simulink library "lib_vehicle_dyn"  (R2024b)
settings: Solver=VariableStepAuto  StartTime=0.0  StopTime=10.0  RelTol=1e-3
undefined symbols (not defined in the file): D
libraries: cstextras x3, simulink x1
settings Model: Creator=simon  LastModifiedBy=simon
settings RTWCC: GPUComputeCapability=3.5

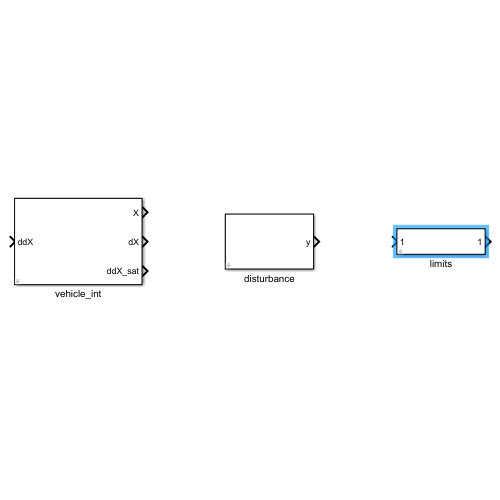
[thumbnail: Simulink's stored preview of the top-level diagram]
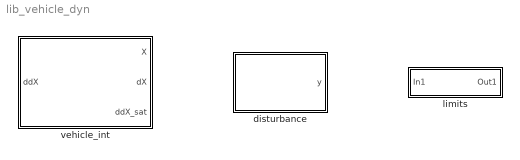
== system lib_vehicle_dyn ==
  disturbance : Subsystem  mask{wn_amp=0, wn_smpl_time=0, wn_gain=0, pg_amp=0, pg_period=0, pg_pw=0, pg_gain=0}
      mask prompts: wn_amp "White noise amplitude"; wn_smpl_time "White noise sampling time"; wn_gain "White noise gain"; pg_amp "Pulse generator amplitude"; pg_period "Pulse generator period"; pg_pw "Pulse generator pulse width [%]"; pg_gain "Pulse generator gain"
      mask DialogControl Control2 Prompt: Disturbance
  limits : Subsystem  mask{satur=0, slew_rate=0, omega=0}
      mask prompts: satur "saturation"
      mask DialogControl Control2 Prompt: Limits
  vehicle_int : Subsystem  mask{x0=0, y0=0, dx0=0, dy0=0, u_sat=0}
      mask DialogControl Control2 Prompt: Vehicle dynamics 2D model

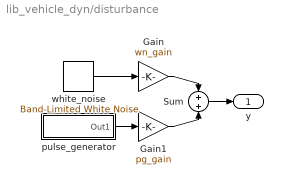
== system lib_vehicle_dyn/disturbance ==
  Gain : Gain  Gain=wn_gain
  Gain1 : Gain  Gain=pg_gain
  Sum : Sum
  pulse_generator : Subsystem
  white_noise : simulink/Sources/Band-Limited White Noise  Cov=wn_amp  Ts=wn_smpl_time  seed=[23341]
  y : Outport
  wires:
  pulse_generator/1(Out1) -> Gain1/1
  white_noise/1 -> Gain/1
  Sum/1 -> y/1
  Gain1/1 -> Sum/2
  Gain/1 -> Sum/1

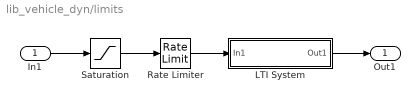
== system lib_vehicle_dyn/limits ==
  In1 : Inport
  LTI System : Subsystem  AncestorBlock=cstblocks/LTI System  BlockChoice=CSS  mask(LTI Block){sys=tf(omega,[1 omega]), IC=[], PadeOrder=0}
      mask prompts: sys "Control:simulink:LTIMaskLabel1"; IC "Control:simulink:LTIMaskLabel2"; PadeOrder "Simulink:blkprm_prompts:TransDelayPadeOrder"
      mask help: Control:simulink:LTIMaskDescription
      mask init:
      | try
      |    % read data to initialize mask variables
      |    [D,Ts,Tdi,Tdo,Tdio,x0,sysname]=...
      |       ltimask('Initialize',gcb,sys,IC);
      |    % update contents
      |    model = bdroot;
      |    df = get_param(model,'dirty');
      |    ltimask('UpdateDiagram',gcb,D,Ts,Tdio,PadeOrder);
      |    try      
      |       % Attempt to modify locked library -> error
      |       % Makes block show ??? when loading CSTBLOCKS
      |       % for the first time
      |       set_param(model,'dirty',df)
      |    end
      | catch ME
      |    sys = [];  IC = [];   sysname = '???';
      |    throw(ME)
      | end
      mask Help: eval('helpview(''control'',''ltisystemblock'');')
      mask Callback sys: ltimask('MaskLTICallback',gcb);
      mask DialogControl sys Prompt: LTI system variable
      mask DialogControl IC Prompt: Initial states (state-space only)
      mask DialogControl PadeOrder Prompt: Pade order (for linearization):
      mask Display: disp(sysname)
  Rate Limiter : RateLimiter  RisingSlewLimit=slew_rate  FallingSlewLimit=-slew_rate  SampleTimeMode=inherited
  Saturation : Saturate  UpperLimit=satur  LowerLimit=-satur
  Out1 : Outport
  wires:
  In1/1 -> Saturation/1
  Saturation/1 -> Rate Limiter/1
  LTI System/1(Out1) -> Out1/1
  Rate Limiter/1 -> LTI System/1(In1)

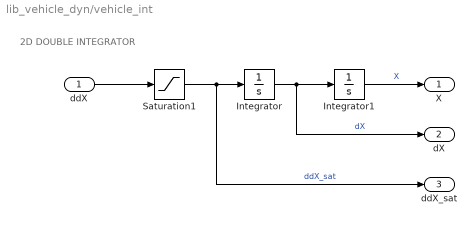
== system lib_vehicle_dyn/vehicle_int ==
  note: 2D DOUBLE INTEGRATOR
  ddX : Inport
  Integrator : Integrator  InitialCondition=[dx0 dy0]
  Integrator1 : Integrator  InitialCondition=[x0 y0]
  Saturation1 : Saturate  UpperLimit=u_sat  LowerLimit=-u_sat
  X : Outport
  dX : Outport  Port=2
  ddX_sat : Outport  Port=3
  wires:
  Saturation1/1 -> ddX_sat/1, Integrator/1  "ddX_sat"
  Integrator/1 -> dX/1, Integrator1/1  "dX"
  ddX/1 -> Saturation1/1
  Integrator1/1 -> X/1  "X"

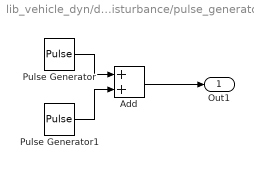
== system lib_vehicle_dyn/disturbance/pulse_generator ==
  Add : Sum
  Pulse Generator : DiscretePulseGenerator  PulseType=Time based  Amplitude=pg_amp  Period=pg_period  PulseWidth=pg_pw
  Pulse Generator1 : DiscretePulseGenerator  PulseType=Time based  Amplitude=-pg_amp  Period=pg_period  PulseWidth=pg_pw  PhaseDelay=pg_period/2
  Out1 : Outport
  wires:
  Pulse Generator1/1 -> Add/2
  Pulse Generator/1 -> Add/1
  Add/1 -> Out1/1

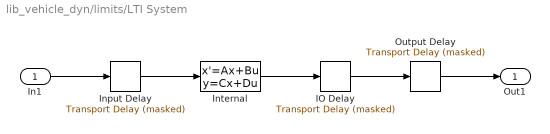
== system lib_vehicle_dyn/limits/LTI System ==
  In1 : Inport
  IO Delay : cstextras/Transport Delay (masked)  Td=Tdio  u0=0  bufsize=1024
  Input Delay : cstextras/Transport Delay (masked)  Td=Tdi  u0=0  bufsize=1024
  Internal : StateSpace  A=D.a  B=D.b  C=D.c  D=D.d
  Output Delay : cstextras/Transport Delay (masked)  Td=Tdo  u0=0  bufsize=1024
  Out1 : Outport  InitialOutput=0  VectorParamsAs1DForOutWhenUnconnected=off
  wires:
  In1/1 -> Input Delay/1
  Output Delay/1 -> Out1/1
  Input Delay/1 -> Internal/1
  Internal/1 -> IO Delay/1
  IO Delay/1 -> Output Delay/1
